simulink model "J2_PMSM_Stage1"  (R2026b)
settings: Solver=ode23t  StopTime=0.02  MaxStep=1e-5  RelTol=1e-6  AbsTol=1e-8
model workspace (MAT data in the model file):
  free_rotor = 0
  p.pp = 8
  p.Rs = 0.04675
  p.Ld = 6.15e-05
  p.Lq = 6.15e-05
  p.Kt = 0.0436218747098
  p.psi = 0.00363515622582
  p.Jm = 1.7e-05
  p.IN = 10.4269458616
  p.nmax_rpm = 6000
  p.Vdc = 24
  p.Vmax = 12.4707658145
  p.Imax = 20.9
  p.Kp = 0.386415896392
  p.Ki = 293.738913111
  p.Kaw = 760.162601626
  p.N = 100
  p.JWG = 7.9e-06
  p.s = -1
  p.Kg = 14000
  p.zeta_g = 0.05
  p.cg = 5.90423576765
  p.J_test = 7.49e-05
libraries: sl_discontinuities x1
settings Model: Creator=rninh  LastModifiedBy=rninh

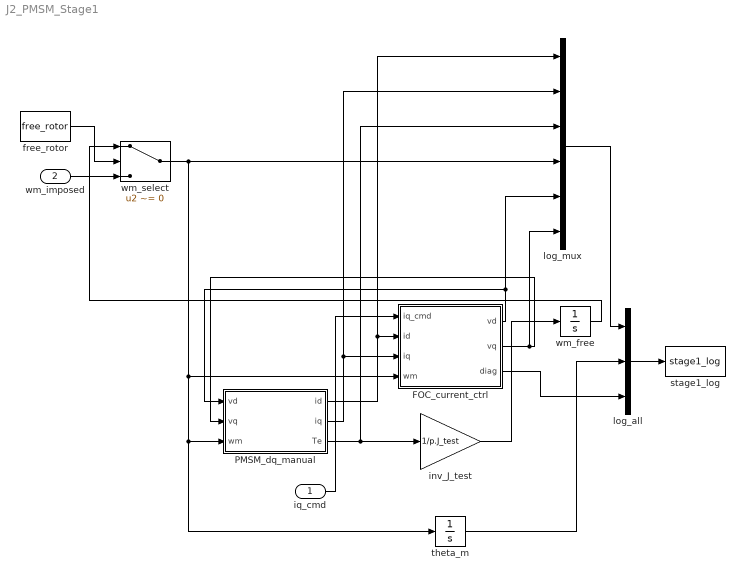
== system J2_PMSM_Stage1 ==
  iq_cmd : Inport  Interpolate=off
  wm_imposed : Inport  Port=2  Interpolate=off
  FOC_current_ctrl : Subsystem
  PMSM_dq_manual : Subsystem
  free_rotor : Constant  Value=free_rotor
  inv_J_test : Gain  Gain=1/p.J_test
  log_all : Mux  Inputs=3
  log_mux : Mux  Inputs=6
  stage1_log : ToWorkspace  VariableName=stage1_log  SaveFormat=Timeseries  SampleTime=-1
  theta_m : Integrator
  wm_free : Integrator
  wm_select : Switch  Criteria=u2 ~= 0  SaturateOnIntegerOverflow=off  InputSameDT=off
  wires:
  wm_free/1 -> wm_select/1
  iq_cmd/1 -> FOC_current_ctrl/1(iq_cmd)
  free_rotor/1 -> wm_select/2
  wm_imposed/1 -> wm_select/3
  PMSM_dq_manual/3(Te) -> log_mux/3, inv_J_test/1
  wm_select/1 -> PMSM_dq_manual/3(wm), theta_m/1, FOC_current_ctrl/4(wm), log_mux/4
  PMSM_dq_manual/2(iq) -> log_mux/2, FOC_current_ctrl/3(iq)
  PMSM_dq_manual/1(id) -> log_mux/1, FOC_current_ctrl/2(id)
  FOC_current_ctrl/1(vd) -> log_mux/5, PMSM_dq_manual/1(vd)
  FOC_current_ctrl/2(vq) -> log_mux/6, PMSM_dq_manual/2(vq)
  FOC_current_ctrl/3(diag) -> log_all/3
  inv_J_test/1 -> wm_free/1
  theta_m/1 -> log_all/2
  log_mux/1 -> log_all/1
  log_all/1 -> stage1_log/1

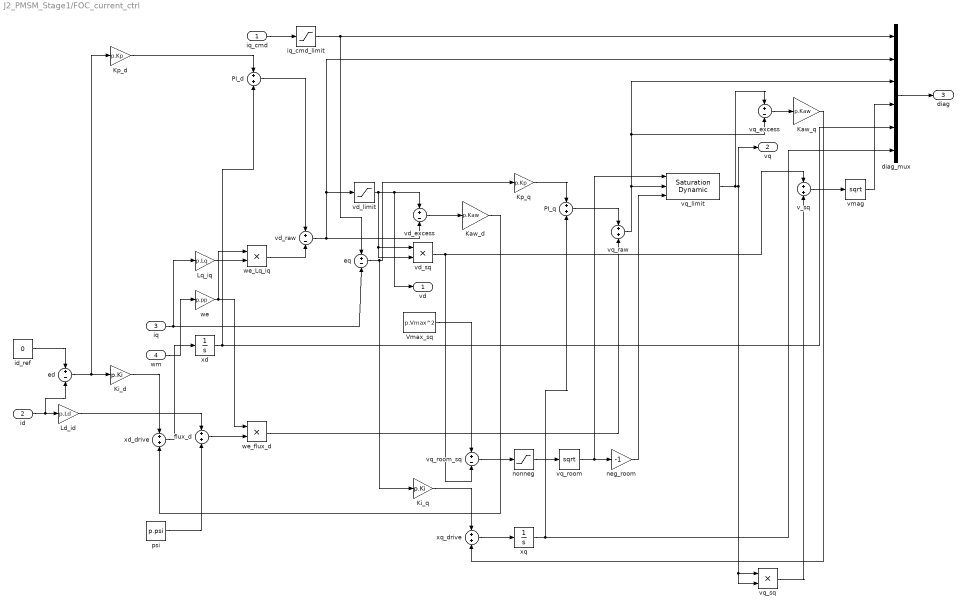
== system J2_PMSM_Stage1/FOC_current_ctrl ==
  iq_cmd : Inport
  id : Inport  Port=2
  iq : Inport  Port=3
  wm : Inport  Port=4
  Kaw_d : Gain  Gain=p.Kaw
  Kaw_q : Gain  Gain=p.Kaw
  Ki_d : Gain  Gain=p.Ki
  Ki_q : Gain  Gain=p.Ki
  Kp_d : Gain  Gain=p.Kp
  Kp_q : Gain  Gain=p.Kp
  Ld_id : Gain  Gain=p.Ld
  Lq_iq : Gain  Gain=p.Lq
  PI_d : Sum
  PI_q : Sum
  Vmax_sq : Constant  Value=p.Vmax^2
  diag_mux : Mux  Inputs=6
  ed : Sum  Inputs=+-
  eq : Sum  Inputs=+-
  flux_d : Sum
  id_ref : Constant  Value=0
  iq_cmd_limit : Saturate  UpperLimit=p.Imax  LowerLimit=-p.Imax
  neg_room : Gain  Gain=-1
  nonneg : Saturate  UpperLimit=inf  LowerLimit=0
  psi : Constant  Value=p.psi
  v_sq : Sum
  vd_excess : Sum  Inputs=+-
  vd_limit : Saturate  UpperLimit=p.Vmax  LowerLimit=-p.Vmax
  vd_raw : Sum  Inputs=+-
  vd_sq : Product
  vmag : Sqrt
  vq_excess : Sum  Inputs=+-
  vq_limit : sl_discontinuities/Saturation Dynamic  OutMin=[]  OutMax=[]  OutDataTypeStr=Inherit: Same as second input  OutDataType=fixdt(1, 16)  OutScaling=2^-10  DoSatur=off
      settings: LibrarySourceBlock=|
      | simulink/Discontinuities/Saturation
      | Dynamic
  vq_raw : Sum
  vq_room : Sqrt
  vq_room_sq : Sum  Inputs=+-
  vq_sq : Product
  we : Gain  Gain=p.pp
  we_Lq_iq : Product
  we_flux_d : Product
  xd : Integrator
  xd_drive : Sum
  xq : Integrator
  xq_drive : Sum
  vd : Outport
  vq : Outport  Port=2
  diag : Outport  Port=3
  wires:
  wm/1 -> we/1
  iq_cmd_limit/1 -> eq/1, diag_mux/1
  id_ref/1 -> ed/1
  id/1 -> ed/2, Ld_id/1
  Kp_d/1 -> PI_d/1
  we/1 -> we_Lq_iq/1, we_flux_d/1
  ed/1 -> Kp_d/1, Ki_d/1
  Ld_id/1 -> flux_d/1
  Ki_d/1 -> xd_drive/1
  iq/1 -> Lq_iq/1, eq/2
  xd_drive/1 -> xd/1
  diag_mux/1 -> diag/1
  vmag/1 -> diag_mux/4
  we_flux_d/1 -> vq_raw/2
  psi/1 -> flux_d/2
  v_sq/1 -> vmag/1
  Lq_iq/1 -> we_Lq_iq/2
  vd_excess/1 -> Kaw_d/1
  xd/1 -> PI_d/2, diag_mux/5
  Kaw_q/1 -> xq_drive/2
  flux_d/1 -> we_flux_d/2
  iq_cmd/1 -> iq_cmd_limit/1
  xq/1 -> PI_q/2, diag_mux/6
  PI_d/1 -> vd_raw/1
  vq_sq/1 -> v_sq/2
  we_Lq_iq/1 -> vd_raw/2
  vd_raw/1 -> diag_mux/2, vd_limit/1, vd_excess/2
  vd_limit/1 -> vd_sq/2, vd_sq/1, vd_excess/1, vd/1
  vq_limit/1 -> vq_sq/1, vq_sq/2, vq/1, vq_excess/1
  eq/1 -> Kp_q/1, Ki_q/1
  vd_sq/1 -> vq_room_sq/2, v_sq/1
  neg_room/1 -> vq_limit/3
  Vmax_sq/1 -> vq_room_sq/1
  Ki_q/1 -> xq_drive/1
  Kaw_d/1 -> xd_drive/2
  vq_room_sq/1 -> nonneg/1
  xq_drive/1 -> xq/1
  Kp_q/1 -> PI_q/1
  vq_raw/1 -> vq_excess/2, diag_mux/3, vq_limit/2
  nonneg/1 -> vq_room/1
  PI_q/1 -> vq_raw/1
  vq_room/1 -> vq_limit/1, neg_room/1
  vq_excess/1 -> Kaw_q/1

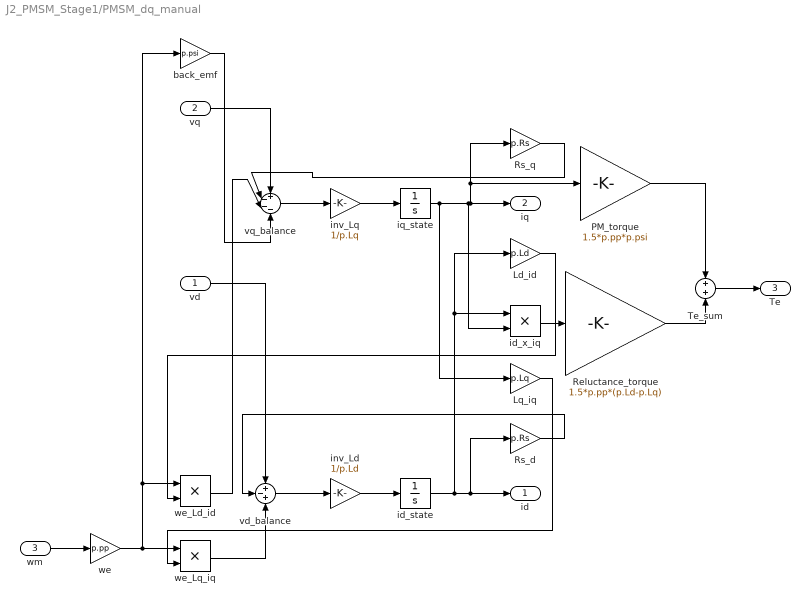
== system J2_PMSM_Stage1/PMSM_dq_manual ==
  vd : Inport
  vq : Inport  Port=2
  wm : Inport  Port=3
  Ld_id : Gain  Gain=p.Ld
  Lq_iq : Gain  Gain=p.Lq
  PM_torque : Gain  Gain=1.5*p.pp*p.psi
  Reluctance_torque : Gain  Gain=1.5*p.pp*(p.Ld-p.Lq)
  Rs_d : Gain  Gain=p.Rs
  Rs_q : Gain  Gain=p.Rs
  Te_sum : Sum
  back_emf : Gain  Gain=p.psi
  id_state : Integrator
  id_x_iq : Product
  inv_Ld : Gain  Gain=1/p.Ld
  inv_Lq : Gain  Gain=1/p.Lq
  iq_state : Integrator
  vd_balance : Sum  Inputs=+-+
  vq_balance : Sum  Inputs=+---
  we : Gain  Gain=p.pp
  we_Ld_id : Product
  we_Lq_iq : Product
  id : Outport
  iq : Outport  Port=2
  Te : Outport  Port=3
  wires:
  Ld_id/1 -> we_Ld_id/2
  id_state/1 -> Rs_d/1, id/1, Ld_id/1, id_x_iq/1
  vq_balance/1 -> inv_Lq/1
  vq/1 -> vq_balance/1
  wm/1 -> we/1
  we/1 -> we_Ld_id/1, back_emf/1, we_Lq_iq/1
  PM_torque/1 -> Te_sum/1
  we_Ld_id/1 -> vq_balance/3
  vd/1 -> vd_balance/1
  back_emf/1 -> vq_balance/4
  Lq_iq/1 -> we_Lq_iq/2
  we_Lq_iq/1 -> vd_balance/3
  Rs_d/1 -> vd_balance/2
  vd_balance/1 -> inv_Ld/1
  inv_Lq/1 -> iq_state/1
  inv_Ld/1 -> id_state/1
  iq_state/1 -> Rs_q/1, PM_torque/1, iq/1, id_x_iq/2, Lq_iq/1
  Rs_q/1 -> vq_balance/2
  id_x_iq/1 -> Reluctance_torque/1
  Te_sum/1 -> Te/1
  Reluctance_torque/1 -> Te_sum/2
